simulink model "hydrofoil_sim"  (R2024b)
settings: Solver=ode45  StartTime=0.0  StopTime=Tstop  MaxStep=0.005  RelTol=1e-6
PostLoadFcn:
  | addpath(fileparts(get_param('hydrofoil_sim', 'FileName'))); hydrofoil_sim_init;
InitFcn:
  | hydrofoil_sim_init;
values from neighbouring files (symbols this model uses):
  A = zeros(4)    [hydrofoil_lin.m]
  act_on = 1    [run_simulink.m]
  B = [0 0; k/p.m; 0 0; k.*x/p.Iy]    [hydrofoil_lin.m]
  ctrl_on = 1    [run_simulink.m]
  dc = design_digital(p, p.Ts_ctrl, 1)    [ctrl_server.m]    (also in design_digital.m = struct('Ts', Ts, 'delay', delay, 'Ad', Ad, 'Bd', Bd,        ; make_paper_figs.m; run_irregular.m; run_observer_compare.m)
  noise_on = 1    [run_simulink.m]
  p = params()    [ctrl_server.m]    (also in make_paper_figs.m; run_digital.m; run_irregular.m; run_lqr.m)
  u0 = (L0./(0.5*p.rho*p.U^2*p.S*K0) - p.CL0)/p.CLa    [hydrofoil_trim.m]    (also in sim_closed_loop.m = u0(:); sim_digital.m = u0(:))
  wave_on = 1    [run_simulink.m]
  wv = wave_irregular(p, 0.15, 3.0, 1)    [make_paper_figs.m]    (also in run_digital.m = wave_params(p); run_irregular.m = wave_irregular(p, seas(2).Hs, seas(2).Tp, 1); run_lqr.m = wave_params(p); run_observer.m = wave_params(p))
settings Model: Creator=lishe  LastModifiedBy=lishe
settings SolverCC: ZeroCrossControl=DisableAll
settings DataIOCC: SaveOutput=off  SaveTime=off

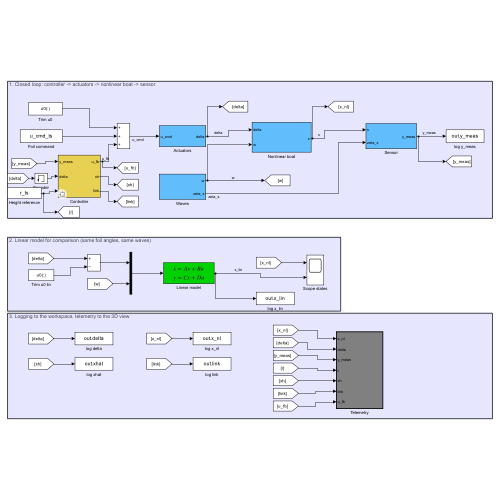
[thumbnail: Simulink's stored preview of the top-level diagram]
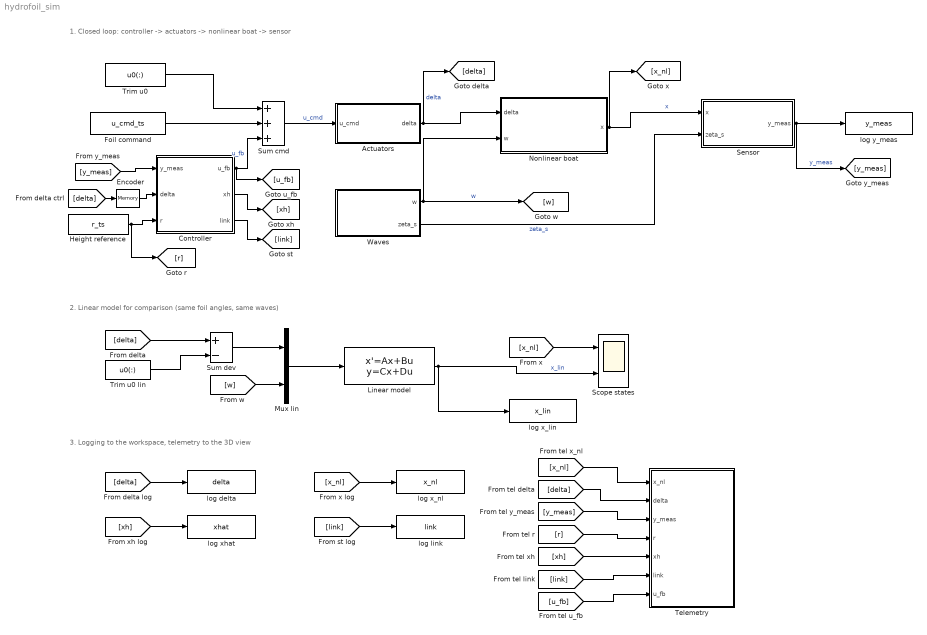
== system hydrofoil_sim ==
  note: 1. Closed loop: controller -> actuators -> nonlinear boat -> sensor
  note: 2. Linear model for comparison (same foil angles, same waves)
  note: 3. Logging to the workspace, telemetry to the 3D view
  Actuators : Subsystem
  Controller : Subsystem  Variant=on
  Encoder : Memory  InitialCondition=u0(:)
  Foil command : FromWorkspace  VariableName=u_cmd_ts  OutputAfterFinalValue=Holding final value
  Height reference : FromWorkspace  VariableName=r_ts  OutputAfterFinalValue=Holding final value
  Linear model : StateSpace  A=A  B=[B E]  C=eye(4)  D=zeros(4,4)  InitialCondition=zeros(4,1)
  Mux lin : Mux  Inputs=2
  Nonlinear boat : Subsystem
  Scope states : Scope  NumInputPorts=2
  Sensor : Subsystem
  Sum cmd : Sum  Inputs=+++
  Sum dev : Sum  Inputs=+-
  Telemetry : Subsystem  TreatAsAtomicUnit=on  SystemSampleTime=p.Ts_ctrl
  Trim u0 : Constant  Value=u0(:)
  Trim u0 lin : Constant  Value=u0(:)
  Waves : Subsystem
  log delta : ToWorkspace  VariableName=delta  SaveFormat=Timeseries  SampleTime=-1
  log link : ToWorkspace  VariableName=link  SaveFormat=Timeseries  SampleTime=-1
  log x_lin : ToWorkspace  VariableName=x_lin  SaveFormat=Timeseries  SampleTime=-1
  log x_nl : ToWorkspace  VariableName=x_nl  SaveFormat=Timeseries  SampleTime=-1
  log xhat : ToWorkspace  VariableName=xhat  SaveFormat=Timeseries  SampleTime=-1
  log y_meas : ToWorkspace  VariableName=y_meas  SaveFormat=Timeseries  SampleTime=-1
  wires:
  Trim u0/1 -> Sum cmd/1
  Foil command/1 -> Sum cmd/2
  [y_meas] -> Controller/1(y_meas)
  [delta] -> Encoder/1
  Encoder/1 -> Controller/2(delta)
  Height reference/1 -> Controller/3(r), [r]
  Controller/1(u_fb) -> Sum cmd/3, [u_fb]  "u_fb"
  Controller/2(xh) -> [xh]
  Controller/3(link) -> [link]
  Sum cmd/1 -> Actuators/1(u_cmd)  "u_cmd"
  Actuators/1(delta) -> Nonlinear boat/1(delta), [delta]  "delta"
  Waves/1(w) -> [w], Nonlinear boat/2(w)  "w"
  Waves/2(zeta_s) -> Sensor/2(zeta_s)  "zeta_s"
  Nonlinear boat/1(x) -> Sensor/1(x), [x_nl]  "x"
  Sensor/1(y_meas) -> log y_meas/1, [y_meas]  "y_meas"
  [delta] -> Sum dev/1
  Trim u0 lin/1 -> Sum dev/2
  Sum dev/1 -> Mux lin/1
  [w] -> Mux lin/2
  Mux lin/1 -> Linear model/1
  Linear model/1 -> Scope states/2, log x_lin/1  "x_lin"
  [x_nl] -> Scope states/1
  [delta] -> log delta/1
  [x_nl] -> log x_nl/1
  [xh] -> log xhat/1
  [link] -> log link/1
  [x_nl] -> Telemetry/1(x_nl)
  [delta] -> Telemetry/2(delta)
  [y_meas] -> Telemetry/3(y_meas)
  [r] -> Telemetry/4(r)
  [xh] -> Telemetry/5(xh)
  [link] -> Telemetry/6(link)
  [u_fb] -> Telemetry/7(u_fb)

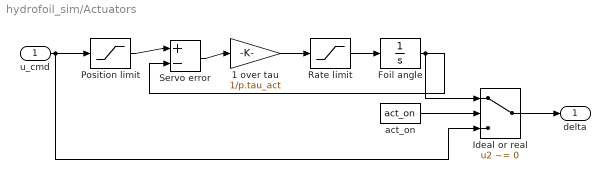
== system hydrofoil_sim/Actuators ==
  u_cmd : Inport
  1 over tau : Gain  Gain=1/p.tau_act
  Foil angle : Integrator  InitialCondition=u0(:)
  Ideal or real : Switch  Criteria=u2 ~= 0  SaturateOnIntegerOverflow=off  InputSameDT=off
  Position limit : Saturate  UpperLimit=p.u_max  LowerLimit=p.u_min
  Rate limit : Saturate  UpperLimit=p.rate_max  LowerLimit=-p.rate_max
  Servo error : Sum  Inputs=+-
  act_on : Constant  Value=act_on
  delta : Outport
  wires:
  u_cmd/1 -> Position limit/1, Ideal or real/3
  Position limit/1 -> Servo error/1
  Servo error/1 -> 1 over tau/1
  1 over tau/1 -> Rate limit/1
  Rate limit/1 -> Foil angle/1
  Foil angle/1 -> Servo error/2, Ideal or real/1
  act_on/1 -> Ideal or real/2
  Ideal or real/1 -> delta/1

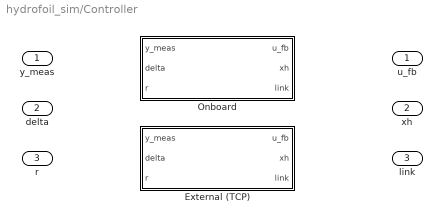
== system hydrofoil_sim/Controller ==
  y_meas : Inport
  delta : Inport  Port=2
  r : Inport  Port=3
  External (TCP) : Subsystem  TreatAsAtomicUnit=on  SystemSampleTime=p.Ts_ctrl  VariantControl=ctrl_ext == 1
  Onboard : Subsystem  TreatAsAtomicUnit=on  SystemSampleTime=p.Ts_ctrl  VariantControl=ctrl_ext == 0
  u_fb : Outport
  xh : Outport  Port=2
  link : Outport  Port=3

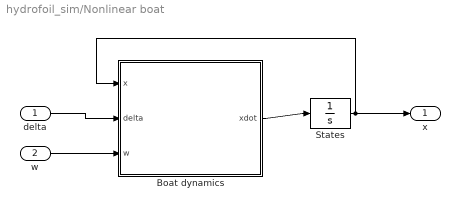
== system hydrofoil_sim/Nonlinear boat ==
  delta : Inport
  w : Inport  Port=2
  Boat dynamics : MATLAB Function  TreatAsAtomicUnit=on
  States : Integrator  InitialCondition=zeros(4,1)
  x : Outport
  wires:
  Boat dynamics/1(xdot) -> States/1
  States/1 -> x/1, Boat dynamics/1(x)
  delta/1 -> Boat dynamics/2(delta)
  w/1 -> Boat dynamics/3(w)

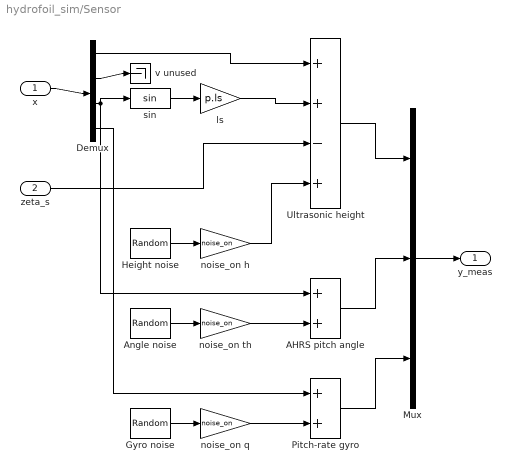
== system hydrofoil_sim/Sensor ==
  x : Inport
  zeta_s : Inport  Port=2
  AHRS pitch angle : Sum
  Angle noise : RandomNumber  Variance=p.sigma_th^2  Seed=3  SampleTime=p.Ts_sens
  Demux : Demux
  Gyro noise : RandomNumber  Variance=p.sigma_q^2  Seed=2  SampleTime=p.Ts_sens
  Height noise : RandomNumber  Variance=p.sigma_y^2  Seed=1  SampleTime=p.Ts_sens
  Mux : Mux  Inputs=3
  Pitch-rate gyro : Sum
  Ultrasonic height : Sum  Inputs=++-+
  ls : Gain  Gain=p.ls
  noise_on h : Gain  Gain=noise_on
  noise_on q : Gain  Gain=noise_on
  noise_on th : Gain  Gain=noise_on
  sin : Trigonometry
  v unused : Terminator
  y_meas : Outport
  wires:
  x/1 -> Demux/1
  Demux/1 -> Ultrasonic height/1
  Demux/2 -> v unused/1
  Demux/3 -> sin/1, AHRS pitch angle/1
  sin/1 -> ls/1
  ls/1 -> Ultrasonic height/2
  zeta_s/1 -> Ultrasonic height/3
  Height noise/1 -> noise_on h/1
  noise_on h/1 -> Ultrasonic height/4
  Angle noise/1 -> noise_on th/1
  noise_on th/1 -> AHRS pitch angle/2
  Demux/4 -> Pitch-rate gyro/1
  Gyro noise/1 -> noise_on q/1
  noise_on q/1 -> Pitch-rate gyro/2
  Ultrasonic height/1 -> Mux/1
  AHRS pitch angle/1 -> Mux/2
  Pitch-rate gyro/1 -> Mux/3
  Mux/1 -> y_meas/1

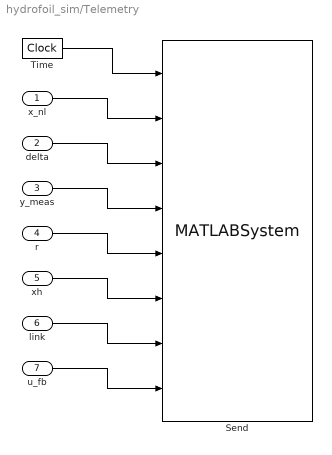
== system hydrofoil_sim/Telemetry ==
  x_nl : Inport
  delta : Inport  Port=2
  y_meas : Inport  Port=3
  r : Inport  Port=4
  xh : Inport  Port=5
  link : Inport  Port=6
  u_fb : Inport  Port=7
  Send : MATLABSystem  System=SilTelemetry  Host=127.0.0.1  Port=5502  Setup=sil_setup  Enabled=viz_on
      mask Type: SilTelemetry
      mask Display:
      | disp('SilTelemetry');
      | port_label('input',1,'t');
      | port_label('input',2,'x');
      | port_label('input',3,'delta');
      | port_label('input',4,'y');
      | port_label('input',5,'r');
      | port_label('input',6,'xh');
      | port_label('input',7,'st');
      | port_label('input',8,'u_fb');
  Time : DigitalClock  SampleTime=p.Ts_ctrl
  wires:
  Time/1 -> Send/1
  x_nl/1 -> Send/2
  delta/1 -> Send/3
  y_meas/1 -> Send/4
  r/1 -> Send/5
  xh/1 -> Send/6
  link/1 -> Send/7
  u_fb/1 -> Send/8

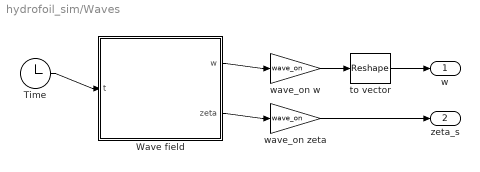
== system hydrofoil_sim/Waves ==
  Time : Clock
  Wave field : MATLAB Function  TreatAsAtomicUnit=on
  to vector : Reshape
  wave_on w : Gain  Gain=wave_on
  wave_on zeta : Gain  Gain=wave_on
  w : Outport
  zeta_s : Outport  Port=2
  wires:
  Time/1 -> Wave field/1(t)
  Wave field/1(w) -> wave_on w/1
  Wave field/2(zeta) -> wave_on zeta/1
  wave_on w/1 -> to vector/1
  to vector/1 -> w/1
  wave_on zeta/1 -> zeta_s/1

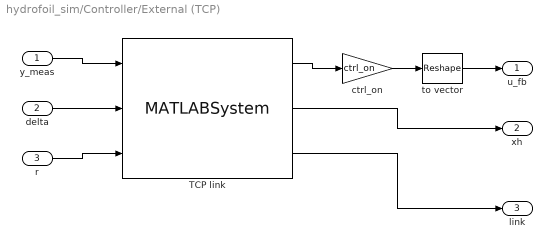
== system hydrofoil_sim/Controller/External (TCP) ==
  y_meas : Inport
  delta : Inport  Port=2
  r : Inport  Port=3
  TCP link : MATLABSystem  System=SilLink  Host=127.0.0.1  Port=5501  Lockstep=sil_lockstep  ExtraMs=sil_extra_ms  JitterMs=sil_jitter_ms
      mask Type: SilLink
      mask Display:
      | disp('SilLink');
      | port_label('input',1,'y');
      | port_label('input',2,'delta');
      | port_label('input',3,'r');
      | port_label('output',1,'u_fb');
      | port_label('output',2,'xh');
      | port_label('output',3,'st');
  ctrl_on : Gain  Gain=ctrl_on
  to vector : Reshape
  u_fb : Outport
  xh : Outport  Port=2
  link : Outport  Port=3
  wires:
  ctrl_on/1 -> to vector/1
  to vector/1 -> u_fb/1
  y_meas/1 -> TCP link/1
  delta/1 -> TCP link/2
  r/1 -> TCP link/3
  TCP link/1 -> ctrl_on/1
  TCP link/2 -> xh/1
  TCP link/3 -> link/1

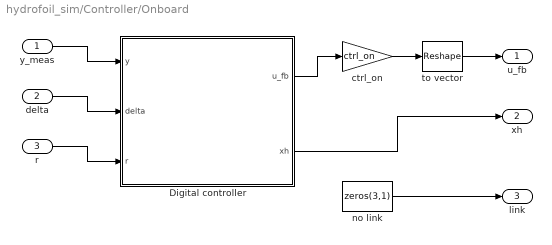
== system hydrofoil_sim/Controller/Onboard ==
  y_meas : Inport
  delta : Inport  Port=2
  r : Inport  Port=3
  Digital controller : MATLAB Function  TreatAsAtomicUnit=on
  ctrl_on : Gain  Gain=ctrl_on
  no link : Constant  Value=zeros(3,1)
  to vector : Reshape
  u_fb : Outport
  xh : Outport  Port=2
  link : Outport  Port=3
  wires:
  ctrl_on/1 -> to vector/1
  to vector/1 -> u_fb/1
  y_meas/1 -> Digital controller/1(y)
  delta/1 -> Digital controller/2(delta)
  r/1 -> Digital controller/3(r)
  Digital controller/1(u_fb) -> ctrl_on/1
  Digital controller/2(xh) -> xh/1
  no link/1 -> link/1

== matlab function hydrofoil_sim/Nonlinear boat/Boat dynamics ==
  data: x input; xdot output; delta input; w input; p parameter
function xdot = boat_dynamics(x, delta, w, p)
% Nonlinear heave/pitch dynamics, see hydrofoil_nl.m
[xdot, ~] = hydrofoil_nl(x, delta, w, p);

== matlab function hydrofoil_sim/Controller/Onboard/Digital controller ==
  data: y input; u_fb output; delta input; r input; xh output; dc parameter; p parameter; u0 parameter
function [u_fb, xh] = digital_controller_block(y, delta, r, dc, p, u0)
% One sample of the 50 Hz controller, see digital_controller.m
[u_fb, xh] = digital_controller(y, delta, r, dc, p, u0);

== matlab function hydrofoil_sim/Waves/Wave field ==
  data: t input; w output; zeta output; wv parameter; p parameter
function [w, zeta] = wave_field(t, wv, p)
% Water velocity at the foils and surface under the sensor, see wave_eval.m
[wr, zeta] = wave_eval(wv, t, p);
w = wr(:);
